simulink model "antenna_dc_fuzzy"  (R2026a)
settings: Solver=ode4  StopTime=48  FixedStep=1e-4
InitFcn:
  | addpath(fileparts(get_param(bdroot,'FileName')));antenna_model_init(bdroot);
model workspace (MAT data in the model file):
  antenna_fis : sugfis (value not decoded)
  dc_cfg.plant.Ra = 1
  dc_cfg.plant.La = 0.005
  dc_cfg.plant.Kt = 0.1
  dc_cfg.plant.Kb = 0.1
  dc_cfg.plant.N = 150
  dc_cfg.plant.J = 7.25
  dc_cfg.plant.B = 3.125
  dc_cfg.plant.Tc = 5
  dc_cfg.plant.epsilon = 0.001
  dc_cfg.Ts = 0.01
  dc_cfg.h = 0.0001
  dc_cfg.duration = 48
  dc_cfg.vmax = 0.48
  dc_cfg.accel = 1.8
  dc_cfg.error_width = 0.08
  dc_cfg.kp_velocity = 6
  dc_cfg.ki_velocity = 35
  dc_cfg.mode = 'fuzzy'
  theta_reference = [0  1.0471975512; 12  2.61799387799; 24  0.523598775598; 36  1.57079632679; 48  1.57079632679]
libraries: fuzblock x1
settings Model: Creator=vutua  LastModifiedBy=vutua

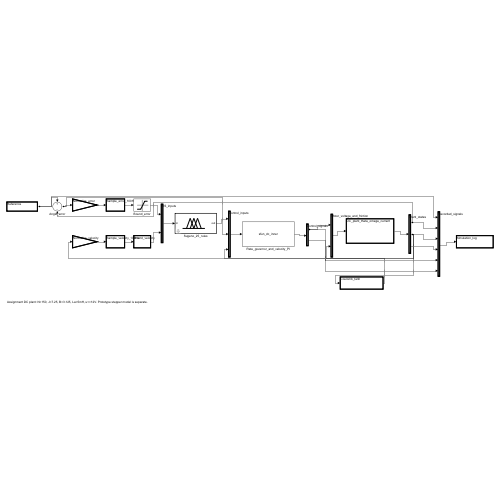
[thumbnail: Simulink's stored preview of the top-level diagram]
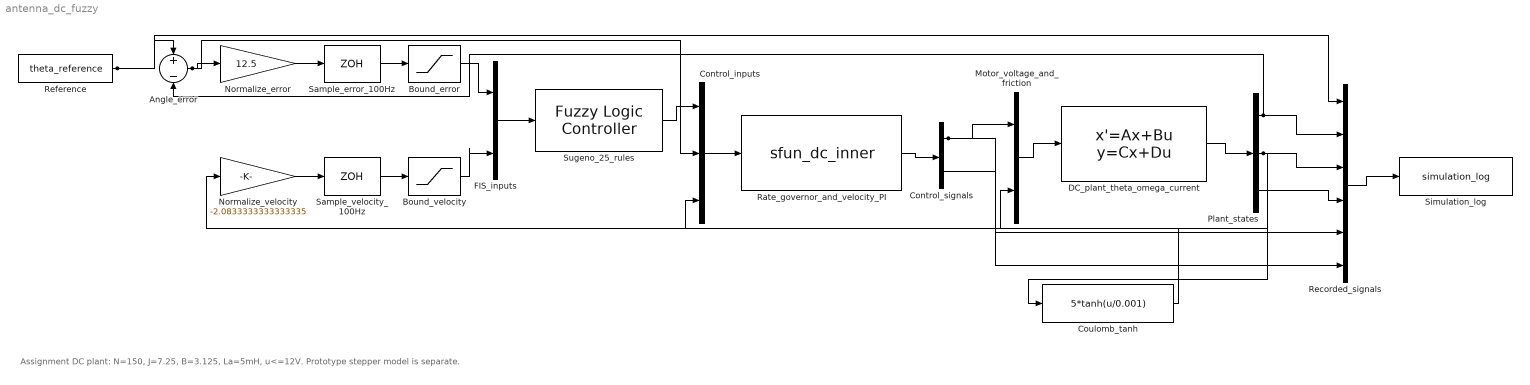
== system antenna_dc_fuzzy ==
  note: Assignment DC plant: N=150, J=7.25, B=3.125, La=5mH, u<=12V. Prototype stepper model is separate.
  Angle_error : Sum  Inputs=+-
  Bound_error : Saturate  UpperLimit=1  LowerLimit=-1
  Bound_velocity : Saturate  UpperLimit=1  LowerLimit=-1
  Control_inputs : Mux  Inputs=3
  Control_signals : Demux  Outputs=2
  Coulomb_tanh : Fcn  Expr=5*tanh(u/0.001)
  DC_plant_theta_omega_current : StateSpace  A=[0 1 0;0 -0.43103448275862066 2.0689655172413794;0 -3000 -200]  B=[0 0;0 -0.13793103448275862;200 0]  C=eye(3)  D=zeros(3,2)  InitialCondition=[0;0;0]
  FIS_inputs : Mux  Inputs=2
  Motor_voltage_and_friction : Mux  Inputs=2
  Normalize_error : Gain  Gain=12.5
  Normalize_velocity : Gain  Gain=-2.0833333333333335
  Plant_states : Demux  Outputs=3
  Rate_governor_and_velocity_PI : M-S-Function  FunctionName=sfun_dc_inner  Parameters=dc_cfg
  Recorded_signals : Mux  Inputs=6
  Reference : FromWorkspace  VariableName=theta_reference  Interpolate=off  OutputAfterFinalValue=Holding final value
  Sample_error_100Hz : ZeroOrderHold  SampleTime=.01
  Sample_velocity_100Hz : ZeroOrderHold  SampleTime=.01
  Simulation_log : ToWorkspace  VariableName=simulation_log  SaveFormat=Structure With Time  SampleTime=-1
  Sugeno_25_rules : fuzblock/Fuzzy Logic  Controller  FIS=antenna_fis  OutputSampleNumber=101  DataType=double  UseLookupTable=off  NumBreakpoints=10  FuzzifiedInputs=off  RuleFiringStrengths=off  RuleOutputs=off  AggregatedOutputs=off  SimulateUsing=Interpreted execution  OutOfRangeInputValueMessage=warning  NoRuleFiredMessage=warning  EmptyOutputFuzzySetMessage=warning
  wires:
  Reference/1 -> Angle_error/1, Recorded_signals/1
  Plant_states/1 -> Angle_error/2, Recorded_signals/2
  Angle_error/1 -> Normalize_error/1, Control_inputs/2
  Normalize_error/1 -> Sample_error_100Hz/1
  Sample_error_100Hz/1 -> Bound_error/1
  Bound_error/1 -> FIS_inputs/1
  Plant_states/2 -> Normalize_velocity/1, Control_inputs/3, Coulomb_tanh/1, Recorded_signals/3
  Normalize_velocity/1 -> Sample_velocity_100Hz/1
  Sample_velocity_100Hz/1 -> Bound_velocity/1
  Bound_velocity/1 -> FIS_inputs/2
  FIS_inputs/1 -> Sugeno_25_rules/1
  Sugeno_25_rules/1 -> Control_inputs/1
  Control_inputs/1 -> Rate_governor_and_velocity_PI/1
  Rate_governor_and_velocity_PI/1 -> Control_signals/1
  Control_signals/1 -> Motor_voltage_and_friction/1, Recorded_signals/5
  Coulomb_tanh/1 -> Motor_voltage_and_friction/2
  Motor_voltage_and_friction/1 -> DC_plant_theta_omega_current/1
  DC_plant_theta_omega_current/1 -> Plant_states/1
  Plant_states/3 -> Recorded_signals/4
  Control_signals/2 -> Recorded_signals/6
  Recorded_signals/1 -> Simulation_log/1
